simulink model "MOBATSim"  (R2020b)
settings: Solver=FixedStepAuto  StartTime=0.0  StopTime=Sim_t  FixedStep=0.01  MinStep=0.01  RelTol=1e-2
values from neighbouring files (symbols this model uses):
  Vehicles = evalin('base','Vehicles')    [I2V.m]    (also in VehicleSensors.m)
undefined symbols (not defined in the file or in its folder): Sim_Ts
libraries: simulink x50, robotalgslib x10, drivingvehiclecontroller x10, mpcadaslib x10, pid_lib x10
(part 7 of 7)

== matlab function MOBATSim/Vehicle Model 8/Longitudinal and Lateral Controllers/Longitudinal Speed Control/Reference Acceleration Generation/Simple Gear Logic ==
  data: speed input; maxAcc output
function maxAcc = fcn(speed)
% Simple gear logic

    if speed < 3
        maxAcc = 6;
    
    elseif speed >= 3 && speed < 6
        maxAcc = 5;
        
    elseif speed >= 6 && speed < 9
        maxAcc = 3.8;
        
    elseif speed >= 9 && speed < 12
        maxAcc = 3;
        
    elseif speed >= 12 && speed < 14
        maxAcc = 2.2;
    else
        % if speed is greater than 14
        maxAcc = 1.4;  
    end

end

== matlab function MOBATSim/Vehicle Model 9/Longitudinal and Lateral Controllers/Longitudinal Speed Control/Reference Acceleration Generation/Simple Gear Logic ==
  data: speed input; maxAcc output
function maxAcc = fcn(speed)
% Simple gear logic

    if speed < 3
        maxAcc = 6;
    
    elseif speed >= 3 && speed < 6
        maxAcc = 5;
        
    elseif speed >= 6 && speed < 9
        maxAcc = 3.8;
        
    elseif speed >= 9 && speed < 12
        maxAcc = 3;
        
    elseif speed >= 12 && speed < 14
        maxAcc = 2.2;
    else
        % if speed is greater than 14
        maxAcc = 1.4;  
    end

end

== matlab function MOBATSim/Vehicle Model 10/Longitudinal and Lateral Controllers/Longitudinal Speed Control/Reference Acceleration Generation/Simple Gear Logic ==
  data: speed input; maxAcc output
function maxAcc = fcn(speed)
% Simple gear logic

    if speed < 3
        maxAcc = 6;
    
    elseif speed >= 3 && speed < 6
        maxAcc = 5;
        
    elseif speed >= 6 && speed < 9
        maxAcc = 3.8;
        
    elseif speed >= 9 && speed < 12
        maxAcc = 3;
        
    elseif speed >= 12 && speed < 14
        maxAcc = 2.2;
    else
        % if speed is greater than 14
        maxAcc = 1.4;  
    end

end

== matlab function MOBATSim/Vehicle Model 2/Longitudinal and Lateral Controllers/Longitudinal Speed Control/Reference Acceleration Generation/Simple Gear Logic ==
  data: speed input; maxAcc output
function maxAcc = fcn(speed)
% Simple gear logic

    if speed < 3
        maxAcc = 6;
    
    elseif speed >= 3 && speed < 6
        maxAcc = 5;
        
    elseif speed >= 6 && speed < 9
        maxAcc = 3.8;
        
    elseif speed >= 9 && speed < 12
        maxAcc = 3;
        
    elseif speed >= 12 && speed < 14
        maxAcc = 2.2;
    else
        % if speed is greater than 14
        maxAcc = 1.4;  
    end

end

== matlab function MOBATSim/Vehicle Model 1/Longitudinal and Lateral Controllers/Longitudinal Speed Control/Reference Acceleration Generation/Simple Gear Logic ==
  data: speed input; maxAcc output
function maxAcc = fcn(speed)
% Simple gear logic

    if speed < 3
        maxAcc = 6;
    
    elseif speed >= 3 && speed < 6
        maxAcc = 5;
        
    elseif speed >= 6 && speed < 9
        maxAcc = 3.8;
        
    elseif speed >= 9 && speed < 12
        maxAcc = 3;
        
    elseif speed >= 12 && speed < 14
        maxAcc = 2.2;
    else
        % if speed is greater than 14
        maxAcc = 1.4;  
    end

end
